simulink model "vienna_rectifier"  (R2026b)
settings: Solver=ode23tb  StopTime=param.sim.simlength  FixedStep=param.glb_time.tc  MaxStep=param.glb_time.tc
values from neighbouring files (symbols this model uses):
  param = struct()    [init_model.m]
undefined symbols (not defined in the file or in its folder): magnitude
libraries: fl_lib x42, nesl_utility x28, discrete_time_low_pass_filter x5, single_phase_transformer_lib x3, threephase_inductor_lib x1, dclink_for_three_levels x1, vienna_rectifier_ideal_switch_based_model x1, three_phase_three_levels_PWM_modulator x1, three_phase_voltage_with_frt_emulator x1
(part 3 of 4)

== system vienna_rectifier/afe_dq_mod1/AFE_control/afe_control/current_ctrl/zero_current_ctrl/zero_sequence_current_ctrl ==
  iz : Inport
  1/Ti : Gain  Gain=param.afe.ctrl.kp_is_z  SaturateOnIntegerOverflow=on  OutDataTypeStr=Inherit: Same as input  ParamDataTypeStr=Inherit: Same as input
  Constant1 : Constant  Value=0
  Gain : Gain
  Saturation : Saturate  UpperLimit=1  LowerLimit=-1
  Sum1 : Sum  Inputs=+++  SaturateOnIntegerOverflow=on
  Sum2 : Sum  Inputs=-+  SaturateOnIntegerOverflow=on
  Sum3 : Sum  Inputs=-+  SaturateOnIntegerOverflow=on
  Unit Delay4 : UnitDelay  SampleTime=-1
  iz_tracking : Scope  NumInputPorts=3
      settings: ActiveDisplayYMinimum=-1  ActiveDisplayYMaximum=1  DataLoggingVariableName=ScopeData8
  kp : Gain  Gain=param.afe.ctrl.ki_is_z*param.glb_time.ts_afe  SaturateOnIntegerOverflow=on  OutDataTypeStr=Inherit: Same as input  ParamDataTypeStr=Inherit: Same as input
  ugamma_afe : Outport
  tag scope: iz_ctrl_out=scoped, iz_pu=scoped, iz_pu_ref=scoped
  wires:
  1/Ti/1 -> Sum1/1, Sum3/1
  kp/1 -> Sum1/2
  Sum3/1 -> Unit Delay4/1
  Unit Delay4/1 -> Sum1/3
  Constant1/1 -> [iz_pu_ref], iz_tracking/1, Sum2/2  "iz_pu_ref"
  iz/1 -> [iz_pu], iz_tracking/2, Sum2/1  "iz_pu"
  Sum2/1 -> kp/1, 1/Ti/1
  Sum1/1 -> Saturation/1
  Saturation/1 -> Gain/1, [iz_ctrl_out], iz_tracking/3, Sum3/2  "iz_ctrl_out"
  Gain/1 -> ugamma_afe/1

== system vienna_rectifier/afe_dq_mod1/AFE_control/afe_control/grid_voltage_phase_lock_loops/DDSRF-PLL/pll_stageA ==
  gamma_grid : Inport
  ug_abc_pu : Inport  Port=2
  Demux : Demux  Outputs=3
  Math Function : Math  Operator=magnitude^2  SignedPower=on
  Math Function1 : Math  Operator=magnitude^2  SignedPower=on
  Reciprocal Sqrt : Sqrt  Operator=rSqrt
  Saturation : Saturate  UpperLimit=inf  LowerLimit=0.02
  Sum : Sum  Inputs=|++
  filter_and_transformation : Subsystem
  sequences : Subsystem
  u_grid_pos_xi : Outport  VectorParamsAs1DForOutWhenUnconnected=off
  u_grid_pos_eta : Outport  Port=2  VectorParamsAs1DForOutWhenUnconnected=off
  tag scope: Vgrid_unorm_ddsrf=scoped
  wires:
  Saturation/1 -> Reciprocal Sqrt/1
  Reciprocal Sqrt/1 -> [Vgrid_unorm_ddsrf]
  Sum/1 -> Saturation/1
  Math Function1/1 -> Sum/2
  Math Function/1 -> Sum/1
  filter_and_transformation/2(ug_beta) -> Math Function1/1, sequences/2(u_grid_beta)
  filter_and_transformation/1(ug_alpha) -> Math Function/1, sequences/1(u_grid_alpha)
  Demux/3 -> filter_and_transformation/3(ug_c)
  Demux/2 -> filter_and_transformation/2(ug_b)
  Demux/1 -> filter_and_transformation/1(ug_a)
  ug_abc_pu/1 -> Demux/1
  sequences/1(u_grid_pos_xi) -> u_grid_pos_xi/1
  sequences/2(u_grid_pos_eta) -> u_grid_pos_eta/1
  gamma_grid/1 -> sequences/3(phase_angle)

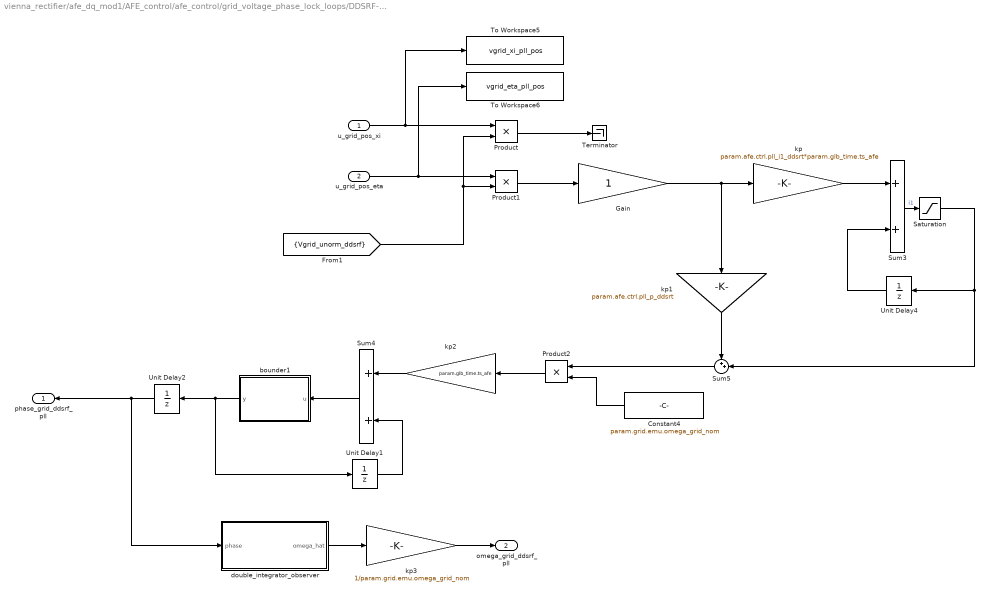
== system vienna_rectifier/afe_dq_mod1/AFE_control/afe_control/grid_voltage_phase_lock_loops/DDSRF-PLL/pll_stageB ==
  u_grid_pos_xi : Inport
  u_grid_pos_eta : Inport  Port=2
  Constant4 : Constant  Value=param.grid.emu.omega_grid_nom
  Gain : Gain
  Product : Product  RndMeth=Zero
  Product1 : Product  RndMeth=Zero
  Product2 : Product  RndMeth=Zero
  Saturation : Saturate  UpperLimit=1.5  LowerLimit=0.5
  Sum3 : Sum  SaturateOnIntegerOverflow=on
  Sum4 : Sum  SaturateOnIntegerOverflow=on
  Sum5 : Sum  Inputs=++|
  Terminator : Terminator
  To Workspace5 : ToWorkspace  VariableName=vgrid_xi_pll_pos  SampleTime=-1
      settings: MaxDataPoints=param.glb_time.Ns_afe
  To Workspace6 : ToWorkspace  VariableName=vgrid_eta_pll_pos  SampleTime=-1
      settings: MaxDataPoints=param.glb_time.Ns_afe
  Unit Delay1 : UnitDelay  SampleTime=-1
  Unit Delay2 : UnitDelay  SampleTime=-1
  Unit Delay4 : UnitDelay  InitialCondition=param.afe.pll.integrator_init  SampleTime=-1
  bounder1 : MATLAB Function  TreatAsAtomicUnit=on
  double_integrator_observer : Subsystem
  kp : Gain  Gain=param.afe.ctrl.pll_i1_ddsrt*param.glb_time.ts_afe  SaturateOnIntegerOverflow=on  OutDataTypeStr=Inherit: Same as input  ParamDataTypeStr=Inherit: Same as input
  kp1 : Gain  Gain=param.afe.ctrl.pll_p_ddsrt  SaturateOnIntegerOverflow=on  OutDataTypeStr=Inherit: Same as input  ParamDataTypeStr=Inherit: Same as input
  kp2 : Gain  Gain=param.glb_time.ts_afe  SaturateOnIntegerOverflow=on  OutDataTypeStr=Inherit: Same as input  ParamDataTypeStr=Inherit: Same as input
  kp3 : Gain  Gain=1/param.grid.emu.omega_grid_nom  SaturateOnIntegerOverflow=on  OutDataTypeStr=Inherit: Same as input  ParamDataTypeStr=Inherit: Same as input
  phase_grid_ddsrf_pll : Outport  VectorParamsAs1DForOutWhenUnconnected=off
  omega_grid_ddsrf_pll : Outport  Port=2  VectorParamsAs1DForOutWhenUnconnected=off
  wires:
  Unit Delay2/1 -> double_integrator_observer/1(phase), phase_grid_ddsrf_pll/1
  kp1/1 -> Sum5/1
  Product2/1 -> kp2/1
  u_grid_pos_eta/1 -> Product1/1, To Workspace6/1
  u_grid_pos_xi/1 -> To Workspace5/1, Product/1
  bounder1/1(y) -> Unit Delay1/1, Unit Delay2/1
  Sum5/1 -> Product2/1
  kp/1 -> Sum3/1
  [Vgrid_unorm_ddsrf] -> Product1/2, Product/2
  Constant4/1 -> Product2/2
  kp2/1 -> Sum4/1
  Sum3/1 -> Saturation/1  "i1"
  Saturation/1 -> Unit Delay4/1, Sum5/2
  Unit Delay1/1 -> Sum4/2
  Sum4/1 -> bounder1/1(u)
  Unit Delay4/1 -> Sum3/2
  double_integrator_observer/1(omega_hat) -> kp3/1
  Product/1 -> Terminator/1
  kp3/1 -> omega_grid_ddsrf_pll/1
  Product1/1 -> Gain/1
  Gain/1 -> kp1/1, kp/1

== system vienna_rectifier/afe_dq_mod1/AFE_control/afe_control/acquisitions/phase_compensation_1/alignment_eval_afe1/pi ==
  u_ref : Inport
  u : Inport  Port=2
  1/Ti : Gain  Gain=kp  SaturateOnIntegerOverflow=on  OutDataTypeStr=Inherit: Same as input  ParamDataTypeStr=Inherit: Same as input
  Saturation : Saturate  UpperLimit=lim_up  LowerLimit=lim_down
  Sum1 : Sum  Inputs=+++  SaturateOnIntegerOverflow=on
  Sum2 : Sum  Inputs=-+  SaturateOnIntegerOverflow=on
  Sum3 : Sum  Inputs=-+  SaturateOnIntegerOverflow=on
  Unit Delay4 : UnitDelay  SampleTime=-1
  kp : Gain  Gain=ki  SaturateOnIntegerOverflow=on  OutDataTypeStr=Inherit: Same as input  ParamDataTypeStr=Inherit: Same as input
  y : Outport
  wires:
  1/Ti/1 -> Sum1/1, Sum3/1
  kp/1 -> Sum1/2
  Sum3/1 -> Unit Delay4/1
  Unit Delay4/1 -> Sum1/3
  u_ref/1 -> Sum2/2
  u/1 -> Sum2/1
  Sum2/1 -> kp/1, 1/Ti/1
  Sum1/1 -> Saturation/1
  Saturation/1 -> Sum3/2, y/1

== system vienna_rectifier/afe_dq_mod1/AFE_control/afe_control/grid_voltage_phase_lock_loops/DDSRF-PLL/pll_stageA/filter_and_transformation ==
  ug_a : Inport
  ug_b : Inport  Port=2
  ug_c : Inport  Port=3
  abc2alphabeta : MATLAB Function  TreatAsAtomicUnit=on
  first_harmonic_tracker : Scope  NumInputPorts=3
      settings: ActiveDisplayYMinimum=-1.2482939809560776  ActiveDisplayYMaximum=1.2484282106161118  DataLoggingVariableName=ScopeData3
  first_harmonic_tracker_phase_u : Subsystem
  first_harmonic_tracker_phase_v : Subsystem
  first_harmonic_tracker_phase_w : Subsystem
  ug_alpha : Outport  VectorParamsAs1DForOutWhenUnconnected=off
  ug_beta : Outport  Port=2  VectorParamsAs1DForOutWhenUnconnected=off
  wires:
  abc2alphabeta/1(alpha) -> ug_alpha/1  "u_grid_alpha"
  abc2alphabeta/2(beta) -> ug_beta/1  "u_grid_beta"
  first_harmonic_tracker_phase_u/1(u_hat) -> first_harmonic_tracker/1, abc2alphabeta/1(a)  "tracker_phase_u"
  first_harmonic_tracker_phase_w/1(u_hat) -> first_harmonic_tracker/3, abc2alphabeta/3(c)  "tracker_phase_w"
  first_harmonic_tracker_phase_v/1(u_hat) -> first_harmonic_tracker/2, abc2alphabeta/2(b)  "tracker_phase_v"
  ug_a/1 -> first_harmonic_tracker_phase_u/1(u)
  ug_b/1 -> first_harmonic_tracker_phase_v/1(u)
  ug_c/1 -> first_harmonic_tracker_phase_w/1(u)

== system vienna_rectifier/afe_dq_mod1/AFE_control/afe_control/grid_voltage_phase_lock_loops/DDSRF-PLL/pll_stageA/sequences ==
  u_grid_alpha : Inport
  u_grid_beta : Inport  Port=2
  phase_angle : Inport  Port=3
  ddsrf : Subsystem
  u_grid_pos_xi : Outport
  u_grid_pos_eta : Outport  Port=2
  wires:
  phase_angle/1 -> ddsrf/3(phase_angle)  "phase_angle"
  u_grid_beta/1 -> ddsrf/2(u_grid_beta)  "u_grid_beta"
  u_grid_alpha/1 -> ddsrf/1(u_grid_alpha)  "u_grid_alpha"
  ddsrf/2(u_grid_pos_eta) -> u_grid_pos_eta/1  "u_grid_pos_eta"
  ddsrf/1(u_grid_pos_xi) -> u_grid_pos_xi/1  "u_grid_pos_xi"

== system vienna_rectifier/afe_dq_mod1/AFE_control/afe_control/grid_voltage_phase_lock_loops/DDSRF-PLL/pll_stageB/double_integrator_observer ==
  phase : Inport
  Gain : Gain  Gain=param.afe.ctrl.di_obs.Ldso  Multiplication=Matrix(K*u)
  Gain1 : Gain  Gain=param.afe.ctrl.di_obs.Adso  Multiplication=Matrix(K*u)
  Gain2 : Gain  Gain=param.afe.ctrl.di_obs.Cso  Multiplication=Matrix(K*u)
  Selector : Selector  InputPortWidth=2  IndexOptions=Index vector (dialog)  Indices=2  OutputSizes=1  RuntimeRangeChecks=off
  Sum : Sum  Inputs=-+|
  Sum1 : Sum  Inputs=|++
  Unit Delay : UnitDelay  SampleTime=-1
  bounder1 : MATLAB Function  TreatAsAtomicUnit=on
  bounder2 : MATLAB Function  TreatAsAtomicUnit=on
  omega_hat : Outport
  wires:
  Gain/1 -> Sum1/1
  Selector/1 -> omega_hat/1
  Gain2/1 -> bounder2/1(u)  "theta_hat"
  Gain1/1 -> Sum1/2
  Sum1/1 -> Unit Delay/1
  Sum/1 -> bounder1/1(u)  "e"
  Unit Delay/1 -> Gain1/1, Selector/1, Gain2/1
  phase/1 -> Sum/2  "phase"
  bounder1/1(y) -> Gain/1  "e_bounded"
  bounder2/1(y) -> Sum/1  "theta_hat_bounded"

== system vienna_rectifier/afe_dq_mod1/AFE_control/afe_control/grid_voltage_phase_lock_loops/DDSRF-PLL/pll_stageA/filter_and_transformation/first_harmonic_tracker_phase_u ==
  u : Inport
  Bus Selector : BusSelector  OutputSignals=output_pu_hat
  C Caller : CCaller  FunctionName=first_harmonic_tracker_process_simulink  PortSpecificationStruct="%)30     .    B \\   8    (     @         %    \"     D    !     0         %  0 \"0    $    _    07)G3F%M90  4&]R=$YA;64 4V-O<&4     26YD97@     5'EP90      4VEZ90      27-';&]B86P   X    P    !@    @    $          4    (     0    ,    !         !   P!O=70 #@   #     &    \"     0         !0    @    !     P    $         $  # &]U=  .    .     8    (    !          %    \"     $    &     0         0  ...(+4988 chars)"
  Constant : Constant  Value=param.glb_time.ts_afe
  Constant1 : Constant  Value=6
  Constant4 : Constant  Value=param.afe.ctrl.fht_grid.omega_fht
  Constant5 : Constant  Value=param.afe.ctrl.fht_grid.delta_fht
  Constant6 : Constant  Value=param.afe.ctrl.fht_grid.Ld_fht(1)
  Constant7 : Constant  Value=param.afe.ctrl.fht_grid.Ld_fht(2)
  Data Type Conversion{1..2,6..9} (6 alike) : DataTypeConversion  OutDataTypeStr=single  SaturateOnIntegerOverflow=off  RndMeth=Floor
  Data Type Conversion3 : DataTypeConversion  OutDataTypeStr=uint8  SaturateOnIntegerOverflow=off  RndMeth=Floor
  Data Type Conversion4 : DataTypeConversion  OutDataTypeStr=double  SaturateOnIntegerOverflow=off  RndMeth=Floor
  Data Type Conversion5 : DataTypeConversion  OutDataTypeStr=uint8  SaturateOnIntegerOverflow=off  RndMeth=Floor
  Step : Step  Time=0.0125  InitialValue=1  FinalValue=0
  u_hat : Outport
  wires:
  Data Type Conversion4/1 -> u_hat/1
  Data Type Conversion3/1 -> C Caller/1
  Data Type Conversion1/1 -> C Caller/3
  Data Type Conversion2/1 -> C Caller/2
  C Caller/1 -> Bus Selector/1
  Bus Selector/1 -> Data Type Conversion4/1  "<output_pu_hat>"
  Step/1 -> Data Type Conversion3/1
  u/1 -> Data Type Conversion2/1
  Constant/1 -> Data Type Conversion1/1
  Constant1/1 -> Data Type Conversion5/1
  Constant4/1 -> Data Type Conversion6/1
  Constant6/1 -> Data Type Conversion8/1
  Constant7/1 -> Data Type Conversion9/1
  Constant5/1 -> Data Type Conversion7/1
  Data Type Conversion5/1 -> C Caller/8
  Data Type Conversion6/1 -> C Caller/4
  Data Type Conversion7/1 -> C Caller/5
  Data Type Conversion8/1 -> C Caller/6
  Data Type Conversion9/1 -> C Caller/7

== system vienna_rectifier/afe_dq_mod1/AFE_control/afe_control/grid_voltage_phase_lock_loops/DDSRF-PLL/pll_stageA/filter_and_transformation/first_harmonic_tracker_phase_v ==
  u : Inport
  Bus Selector : BusSelector  OutputSignals=output_pu_hat
  C Caller : CCaller  FunctionName=first_harmonic_tracker_process_simulink  PortSpecificationStruct="%)30     .    B \\   8    (     @         %    \"     D    !     0         %  0 \"0    $    _    07)G3F%M90  4&]R=$YA;64 4V-O<&4     26YD97@     5'EP90      4VEZ90      27-';&]B86P   X    P    !@    @    $          4    (     0    ,    !         !   P!O=70 #@   #     &    \"     0         !0    @    !     P    $         $  # &]U=  .    .     8    (    !          %    \"     $    &     0         0  ...(+4988 chars)"
  Constant : Constant  Value=param.glb_time.ts_afe
  Constant1 : Constant  Value=8
  Constant4 : Constant  Value=param.afe.ctrl.fht_grid.omega_fht
  Constant5 : Constant  Value=param.afe.ctrl.fht_grid.delta_fht
  Constant6 : Constant  Value=param.afe.ctrl.fht_grid.Ld_fht(1)
  Constant7 : Constant  Value=param.afe.ctrl.fht_grid.Ld_fht(2)
  Data Type Conversion{1..2,6..9} (6 alike) : DataTypeConversion  OutDataTypeStr=single  SaturateOnIntegerOverflow=off  RndMeth=Floor
  Data Type Conversion3 : DataTypeConversion  OutDataTypeStr=uint8  SaturateOnIntegerOverflow=off  RndMeth=Floor
  Data Type Conversion4 : DataTypeConversion  OutDataTypeStr=double  SaturateOnIntegerOverflow=off  RndMeth=Floor
  Data Type Conversion5 : DataTypeConversion  OutDataTypeStr=uint8  SaturateOnIntegerOverflow=off  RndMeth=Floor
  Step : Step  Time=0.0125  InitialValue=1  FinalValue=0
  u_hat : Outport
  wires:
  Data Type Conversion9/1 -> C Caller/7
  Data Type Conversion8/1 -> C Caller/6
  Data Type Conversion7/1 -> C Caller/5
  Data Type Conversion6/1 -> C Caller/4
  Data Type Conversion5/1 -> C Caller/8
  Constant5/1 -> Data Type Conversion7/1
  Constant7/1 -> Data Type Conversion9/1
  Constant6/1 -> Data Type Conversion8/1
  Constant4/1 -> Data Type Conversion6/1
  Constant1/1 -> Data Type Conversion5/1
  Constant/1 -> Data Type Conversion1/1
  u/1 -> Data Type Conversion2/1
  Step/1 -> Data Type Conversion3/1
  Bus Selector/1 -> Data Type Conversion4/1  "<output_pu_hat>"
  C Caller/1 -> Bus Selector/1
  Data Type Conversion2/1 -> C Caller/2
  Data Type Conversion1/1 -> C Caller/3
  Data Type Conversion3/1 -> C Caller/1
  Data Type Conversion4/1 -> u_hat/1

== system vienna_rectifier/afe_dq_mod1/AFE_control/afe_control/grid_voltage_phase_lock_loops/DDSRF-PLL/pll_stageA/filter_and_transformation/first_harmonic_tracker_phase_w ==
  u : Inport
  Bus Selector : BusSelector  OutputSignals=output_pu_hat
  C Caller : CCaller  FunctionName=first_harmonic_tracker_process_simulink  PortSpecificationStruct="%)30     .    B \\   8    (     @         %    \"     D    !     0         %  0 \"0    $    _    07)G3F%M90  4&]R=$YA;64 4V-O<&4     26YD97@     5'EP90      4VEZ90      27-';&]B86P   X    P    !@    @    $          4    (     0    ,    !         !   P!O=70 #@   #     &    \"     0         !0    @    !     P    $         $  # &]U=  .    .     8    (    !          %    \"     $    &     0         0  ...(+4988 chars)"
  Constant : Constant  Value=param.glb_time.ts_afe
  Constant1 : Constant  Value=10
  Constant4 : Constant  Value=param.afe.ctrl.fht_grid.omega_fht
  Constant5 : Constant  Value=param.afe.ctrl.fht_grid.delta_fht
  Constant6 : Constant  Value=param.afe.ctrl.fht_grid.Ld_fht(1)
  Constant7 : Constant  Value=param.afe.ctrl.fht_grid.Ld_fht(2)
  Data Type Conversion{1..2,6..9} (6 alike) : DataTypeConversion  OutDataTypeStr=single  SaturateOnIntegerOverflow=off  RndMeth=Floor
  Data Type Conversion3 : DataTypeConversion  OutDataTypeStr=uint8  SaturateOnIntegerOverflow=off  RndMeth=Floor
  Data Type Conversion4 : DataTypeConversion  OutDataTypeStr=double  SaturateOnIntegerOverflow=off  RndMeth=Floor
  Data Type Conversion5 : DataTypeConversion  OutDataTypeStr=uint8  SaturateOnIntegerOverflow=off  RndMeth=Floor
  Step : Step  Time=0.0125  InitialValue=1  FinalValue=0
  u_hat : Outport
  wires:
  Data Type Conversion4/1 -> u_hat/1
  Data Type Conversion3/1 -> C Caller/1
  Data Type Conversion1/1 -> C Caller/3
  Data Type Conversion2/1 -> C Caller/2
  C Caller/1 -> Bus Selector/1
  Bus Selector/1 -> Data Type Conversion4/1  "<output_pu_hat>"
  Step/1 -> Data Type Conversion3/1
  u/1 -> Data Type Conversion2/1
  Constant/1 -> Data Type Conversion1/1
  Constant1/1 -> Data Type Conversion5/1
  Constant4/1 -> Data Type Conversion6/1
  Constant6/1 -> Data Type Conversion8/1
  Constant7/1 -> Data Type Conversion9/1
  Constant5/1 -> Data Type Conversion7/1
  Data Type Conversion5/1 -> C Caller/8
  Data Type Conversion6/1 -> C Caller/4
  Data Type Conversion7/1 -> C Caller/5
  Data Type Conversion8/1 -> C Caller/6
  Data Type Conversion9/1 -> C Caller/7

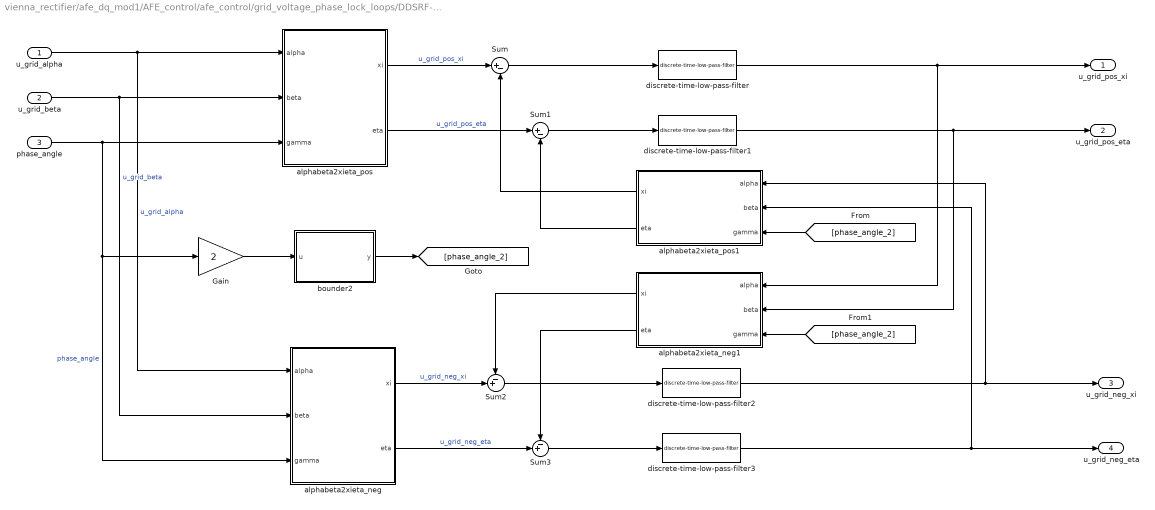
== system vienna_rectifier/afe_dq_mod1/AFE_control/afe_control/grid_voltage_phase_lock_loops/DDSRF-PLL/pll_stageA/sequences/ddsrf ==
  u_grid_alpha : Inport
  u_grid_beta : Inport  Port=2
  phase_angle : Inport  Port=3
  Gain : Gain  Gain=2
  Sum : Sum  Inputs=|+-
  Sum1 : Sum  Inputs=|+-
  Sum2 : Sum  Inputs=-+|
  Sum3 : Sum  Inputs=-+|
  alphabeta2xieta_neg : MATLAB Function  TreatAsAtomicUnit=on
  alphabeta2xieta_neg1 : MATLAB Function  TreatAsAtomicUnit=on
  alphabeta2xieta_pos : MATLAB Function  TreatAsAtomicUnit=on
  alphabeta2xieta_pos1 : MATLAB Function  TreatAsAtomicUnit=on
  bounder2 : MATLAB Function  TreatAsAtomicUnit=on
  discrete-time-low-pass-filter{,1..3} (4 alike) : discrete_time_low_pass_filter/discrete-time-low-pass-filter  tau=param.afe.ctrl.tau_ddsrf  ts=param.glb_time.ts_afe
  u_grid_pos_xi : Outport
  u_grid_pos_eta : Outport  Port=2
  u_grid_neg_xi : Outport  Port=3
  u_grid_neg_eta : Outport  Port=4
  wires:
  phase_angle/1 -> alphabeta2xieta_pos/3(gamma), alphabeta2xieta_neg/3(gamma), Gain/1  "phase_angle"
  u_grid_beta/1 -> alphabeta2xieta_pos/2(beta), alphabeta2xieta_neg/2(beta)  "u_grid_beta"
  u_grid_alpha/1 -> alphabeta2xieta_pos/1(alpha), alphabeta2xieta_neg/1(alpha)  "u_grid_alpha"
  alphabeta2xieta_pos/1(xi) -> Sum/1  "u_grid_pos_xi"
  Sum/1 -> discrete-time-low-pass-filter/1
  alphabeta2xieta_pos/2(eta) -> Sum1/1  "u_grid_pos_eta"
  Sum1/1 -> discrete-time-low-pass-filter1/1
  alphabeta2xieta_neg/1(xi) -> Sum2/2  "u_grid_neg_xi"
  Sum2/1 -> discrete-time-low-pass-filter2/1
  Sum3/1 -> discrete-time-low-pass-filter3/1
  alphabeta2xieta_neg/2(eta) -> Sum3/2  "u_grid_neg_eta"
  Gain/1 -> bounder2/1(u)
  discrete-time-low-pass-filter/1 -> u_grid_pos_xi/1, alphabeta2xieta_neg1/1(alpha)
  discrete-time-low-pass-filter1/1 -> u_grid_pos_eta/1, alphabeta2xieta_neg1/2(beta)
  discrete-time-low-pass-filter2/1 -> u_grid_neg_xi/1, alphabeta2xieta_pos1/1(alpha)
  discrete-time-low-pass-filter3/1 -> u_grid_neg_eta/1, alphabeta2xieta_pos1/2(beta)
  bounder2/1(y) -> [phase_angle_2]
  [phase_angle_2] -> alphabeta2xieta_pos1/3(gamma)
  [phase_angle_2] -> alphabeta2xieta_neg1/3(gamma)
  alphabeta2xieta_pos1/1(xi) -> Sum/2
  alphabeta2xieta_pos1/2(eta) -> Sum1/2
  alphabeta2xieta_neg1/1(xi) -> Sum2/1
  alphabeta2xieta_neg1/2(eta) -> Sum3/1

== matlab function vienna_rectifier/afe_dq_mod1/AFE_control/afe_control/current_ctrl/xi_eta_to_alpha_beta ==
  data: xi input; alpha output; eta input; phase input; beta output
function [alpha,beta] = xi_eta_to_alpha_beta(xi,eta,phase)

    alpha = xi*cos(phase) - eta*sin(phase);
    beta  = xi*sin(phase) + eta*cos(phase);

end

== matlab function vienna_rectifier/afe_dq_mod1/AFE_control/afe_control/grid_voltage_phase_lock_loops/DDSRF-PLL/pll_stageA/sequences/ddsrf/alphabeta2xieta_neg1 ==
  data: alpha input; xi output; beta input; gamma input; eta output
function [xi,eta] = alphabeta2xieta_neg(alpha,beta,gamma)

    xi  = alpha*cos(gamma) - beta*sin(gamma);
    eta = alpha*sin(gamma) + beta*cos(gamma);

end

== matlab function vienna_rectifier/afe_dq_mod1/AFE_control/afe_control/grid_voltage_phase_lock_loops/DDSRF-PLL/pll_stageA/sequences/ddsrf/alphabeta2xieta_pos ==
  data: alpha input; xi output; beta input; gamma input; eta output
function [xi,eta] = alphabeta2xieta_pos(alpha,beta,gamma)

    xi  =  alpha*cos(gamma) + beta*sin(gamma);
    eta = -alpha*sin(gamma) + beta*cos(gamma);

end

== matlab function vienna_rectifier/afe_dq_mod1/AFE_control/afe_control/grid_voltage_phase_lock_loops/DDSRF-PLL/pll_stageA/sequences/ddsrf/alphabeta2xieta_pos1 ==
  data: alpha input; xi output; beta input; gamma input; eta output
function [xi,eta] = alphabeta2xieta_pos(alpha,beta,gamma)

    xi  =  alpha*cos(gamma) + beta*sin(gamma);
    eta = -alpha*sin(gamma) + beta*cos(gamma);

end

== matlab function vienna_rectifier/afe_dq_mod1/AFE_control/afe_control/grid_voltage_phase_lock_loops/DDSRF-PLL/pll_stageA/sequences/ddsrf/bounder2 ==
  data: u input; y output
function y = bounder(u)
    
    y = -pi + mod(u+3*pi,2*pi);
    % y = mod(u, 2*pi);
    
end

== matlab function vienna_rectifier/afe_dq_mod1/AFE_control/afe_control/grid_voltage_phase_lock_loops/DDSRF-PLL/pll_stageB/bounder1 ==
  data: u input; y output
function y = bounder(u)
    y = -pi + mod(u+3*pi,2*pi);
end

== matlab function vienna_rectifier/afe_dq_mod1/rectifier/deadtime_generator_for_ttype/dead_time_generator_cmos_simulink_phu/dead_time_leg_generator_1/MATLAB Function ==
  data: u input; y output; Vpos_rail_dtg parameter
function y = not_cmos(u, Vpos_rail_dtg)

vth = Vpos_rail_dtg/2;

if u > vth
    y = 0;
else
    y = Vpos_rail_dtg;
end

== matlab function vienna_rectifier/afe_dq_mod1/rectifier/deadtime_generator_for_ttype/dead_time_generator_cmos_simulink_phu/dead_time_leg_generator_1/MATLAB Function1 ==
  data: u1 input; u2 input; y output; Vpos_rail_dtg parameter
function y = and_cmos(u1, u2, Vpos_rail_dtg)

vth = Vpos_rail_dtg/2;

if (u1 > vth && u2 > vth)
    y = Vpos_rail_dtg;
else
    y = 0;
end

== matlab function vienna_rectifier/afe_dq_mod1/rectifier/deadtime_generator_for_ttype/dead_time_generator_cmos_simulink_phu/dead_time_leg_generator_1/MATLAB Function2 ==
  data: u input; y output; Vpos_rail_dtg parameter
function y = not_cmos(u, Vpos_rail_dtg)

vth = Vpos_rail_dtg/2;

if u > vth
    y = 0;
else
    y = Vpos_rail_dtg;
end

== matlab function vienna_rectifier/afe_dq_mod1/rectifier/deadtime_generator_for_ttype/dead_time_generator_cmos_simulink_phu/dead_time_leg_generator_1/MATLAB Function3 ==
  data: u input; y output; Vpos_rail_dtg parameter
function y = not_cmos(u, Vpos_rail_dtg)

vth = Vpos_rail_dtg/2;

if u > vth
    y = 0;
else
    y = Vpos_rail_dtg;
end

== matlab function vienna_rectifier/afe_dq_mod1/rectifier/deadtime_generator_for_ttype/dead_time_generator_cmos_simulink_phu/dead_time_leg_generator_1/MATLAB Function4 ==
  data: u1 input; u2 input; y output; Vpos_rail_dtg parameter
function y = and_cmos(u1, u2, Vpos_rail_dtg)

vth = Vpos_rail_dtg/2;

if (u1 > vth && u2 > vth)
    y = Vpos_rail_dtg;
else
    y = 0;
end

== matlab function vienna_rectifier/afe_dq_mod1/rectifier/deadtime_generator_for_ttype/dead_time_generator_cmos_simulink_phu/dead_time_leg_generator_1/MATLAB Function5 ==
  data: u1 input; u2 input; y output; Vpos_rail_dtg parameter
function y = and_cmos(u1, u2, Vpos_rail_dtg)

vth = Vpos_rail_dtg/2;

if (u1 > vth && u2 > vth)
    y = Vpos_rail_dtg;
else
    y = 0;
end

== matlab function vienna_rectifier/afe_dq_mod1/rectifier/deadtime_generator_for_ttype/dead_time_generator_cmos_simulink_phu/dead_time_leg_generator_1/MATLAB Function6 ==
  data: u input; y output; Vpos_rail_dtg parameter
function y = not_cmos(u, Vpos_rail_dtg)

vth = Vpos_rail_dtg/2;

if u > vth
    y = 0;
else
    y = Vpos_rail_dtg;
end

== matlab function vienna_rectifier/afe_dq_mod1/rectifier/deadtime_generator_for_ttype/dead_time_generator_cmos_simulink_phu/dead_time_leg_generator_1/MATLAB Function7 ==
  data: u input; y output; Vpos_rail_dtg parameter
function y = not_cmos(u, Vpos_rail_dtg)

vth = Vpos_rail_dtg/2;

if u > vth
    y = 0;
else
    y = Vpos_rail_dtg;
end

== matlab function vienna_rectifier/afe_dq_mod1/rectifier/deadtime_generator_for_ttype/dead_time_generator_cmos_simulink_phu/dead_time_leg_generator_1/MATLAB Function8 ==
  data: u input; y output; Vpos_rail_dtg parameter
function y = not_cmos(u, Vpos_rail_dtg)

vth = Vpos_rail_dtg/2;

if u > vth
    y = 0;
else
    y = Vpos_rail_dtg;
end

== matlab function vienna_rectifier/afe_dq_mod1/rectifier/deadtime_generator_for_ttype/dead_time_generator_cmos_simulink_phu/dead_time_leg_generator_1/MATLAB Function9 ==
  data: u1 input; u2 input; y output; Vpos_rail_dtg parameter
function y = and_cmos(u1, u2, Vpos_rail_dtg)

vth = Vpos_rail_dtg/2;

if (u1 > vth && u2 > vth)
    y = Vpos_rail_dtg;
else
    y = 0;
end

== matlab function vienna_rectifier/afe_dq_mod1/rectifier/deadtime_generator_for_ttype/dead_time_generator_cmos_simulink_phv/dead_time_leg_generator_1/MATLAB Function ==
  data: u input; y output; Vpos_rail_dtg parameter
function y = not_cmos(u, Vpos_rail_dtg)

vth = Vpos_rail_dtg/2;

if u > vth
    y = 0;
else
    y = Vpos_rail_dtg;
end

== matlab function vienna_rectifier/afe_dq_mod1/rectifier/deadtime_generator_for_ttype/dead_time_generator_cmos_simulink_phv/dead_time_leg_generator_1/MATLAB Function1 ==
  data: u1 input; u2 input; y output; Vpos_rail_dtg parameter
function y = and_cmos(u1, u2, Vpos_rail_dtg)

vth = Vpos_rail_dtg/2;

if (u1 > vth && u2 > vth)
    y = Vpos_rail_dtg;
else
    y = 0;
end

== matlab function vienna_rectifier/afe_dq_mod1/rectifier/deadtime_generator_for_ttype/dead_time_generator_cmos_simulink_phv/dead_time_leg_generator_1/MATLAB Function2 ==
  data: u input; y output; Vpos_rail_dtg parameter
function y = not_cmos(u, Vpos_rail_dtg)

vth = Vpos_rail_dtg/2;

if u > vth
    y = 0;
else
    y = Vpos_rail_dtg;
end

== matlab function vienna_rectifier/afe_dq_mod1/rectifier/deadtime_generator_for_ttype/dead_time_generator_cmos_simulink_phv/dead_time_leg_generator_1/MATLAB Function3 ==
  data: u input; y output; Vpos_rail_dtg parameter
function y = not_cmos(u, Vpos_rail_dtg)

vth = Vpos_rail_dtg/2;

if u > vth
    y = 0;
else
    y = Vpos_rail_dtg;
end

== matlab function vienna_rectifier/afe_dq_mod1/rectifier/deadtime_generator_for_ttype/dead_time_generator_cmos_simulink_phv/dead_time_leg_generator_1/MATLAB Function4 ==
  data: u1 input; u2 input; y output; Vpos_rail_dtg parameter
function y = and_cmos(u1, u2, Vpos_rail_dtg)

vth = Vpos_rail_dtg/2;

if (u1 > vth && u2 > vth)
    y = Vpos_rail_dtg;
else
    y = 0;
end

== matlab function vienna_rectifier/afe_dq_mod1/rectifier/deadtime_generator_for_ttype/dead_time_generator_cmos_simulink_phv/dead_time_leg_generator_1/MATLAB Function5 ==
  data: u1 input; u2 input; y output; Vpos_rail_dtg parameter
function y = and_cmos(u1, u2, Vpos_rail_dtg)

vth = Vpos_rail_dtg/2;

if (u1 > vth && u2 > vth)
    y = Vpos_rail_dtg;
else
    y = 0;
end

== matlab function vienna_rectifier/afe_dq_mod1/rectifier/deadtime_generator_for_ttype/dead_time_generator_cmos_simulink_phv/dead_time_leg_generator_1/MATLAB Function6 ==
  data: u input; y output; Vpos_rail_dtg parameter
function y = not_cmos(u, Vpos_rail_dtg)

vth = Vpos_rail_dtg/2;

if u > vth
    y = 0;
else
    y = Vpos_rail_dtg;
end

== matlab function vienna_rectifier/afe_dq_mod1/rectifier/deadtime_generator_for_ttype/dead_time_generator_cmos_simulink_phv/dead_time_leg_generator_1/MATLAB Function7 ==
  data: u input; y output; Vpos_rail_dtg parameter
function y = not_cmos(u, Vpos_rail_dtg)

vth = Vpos_rail_dtg/2;

if u > vth
    y = 0;
else
    y = Vpos_rail_dtg;
end

== matlab function vienna_rectifier/afe_dq_mod1/rectifier/deadtime_generator_for_ttype/dead_time_generator_cmos_simulink_phv/dead_time_leg_generator_1/MATLAB Function8 ==
  data: u input; y output; Vpos_rail_dtg parameter
function y = not_cmos(u, Vpos_rail_dtg)

vth = Vpos_rail_dtg/2;

if u > vth
    y = 0;
else
    y = Vpos_rail_dtg;
end

== matlab function vienna_rectifier/afe_dq_mod1/rectifier/deadtime_generator_for_ttype/dead_time_generator_cmos_simulink_phv/dead_time_leg_generator_1/MATLAB Function9 ==
  data: u1 input; u2 input; y output; Vpos_rail_dtg parameter
function y = and_cmos(u1, u2, Vpos_rail_dtg)

vth = Vpos_rail_dtg/2;

if (u1 > vth && u2 > vth)
    y = Vpos_rail_dtg;
else
    y = 0;
end

== matlab function vienna_rectifier/afe_dq_mod1/rectifier/deadtime_generator_for_ttype/dead_time_generator_cmos_simulink_phw/dead_time_leg_generator_1/MATLAB Function ==
  data: u input; y output; Vpos_rail_dtg parameter
function y = not_cmos(u, Vpos_rail_dtg)

vth = Vpos_rail_dtg/2;

if u > vth
    y = 0;
else
    y = Vpos_rail_dtg;
end

== matlab function vienna_rectifier/afe_dq_mod1/rectifier/deadtime_generator_for_ttype/dead_time_generator_cmos_simulink_phw/dead_time_leg_generator_1/MATLAB Function1 ==
  data: u1 input; u2 input; y output; Vpos_rail_dtg parameter
function y = and_cmos(u1, u2, Vpos_rail_dtg)

vth = Vpos_rail_dtg/2;

if (u1 > vth && u2 > vth)
    y = Vpos_rail_dtg;
else
    y = 0;
end

== matlab function vienna_rectifier/afe_dq_mod1/rectifier/deadtime_generator_for_ttype/dead_time_generator_cmos_simulink_phw/dead_time_leg_generator_1/MATLAB Function2 ==
  data: u input; y output; Vpos_rail_dtg parameter
function y = not_cmos(u, Vpos_rail_dtg)

vth = Vpos_rail_dtg/2;

if u > vth
    y = 0;
else
    y = Vpos_rail_dtg;
end

== matlab function vienna_rectifier/afe_dq_mod1/rectifier/deadtime_generator_for_ttype/dead_time_generator_cmos_simulink_phw/dead_time_leg_generator_1/MATLAB Function3 ==
  data: u input; y output; Vpos_rail_dtg parameter
function y = not_cmos(u, Vpos_rail_dtg)

vth = Vpos_rail_dtg/2;

if u > vth
    y = 0;
else
    y = Vpos_rail_dtg;
end

== matlab function vienna_rectifier/afe_dq_mod1/rectifier/deadtime_generator_for_ttype/dead_time_generator_cmos_simulink_phw/dead_time_leg_generator_1/MATLAB Function4 ==
  data: u1 input; u2 input; y output; Vpos_rail_dtg parameter
function y = and_cmos(u1, u2, Vpos_rail_dtg)

vth = Vpos_rail_dtg/2;

if (u1 > vth && u2 > vth)
    y = Vpos_rail_dtg;
else
    y = 0;
end

== matlab function vienna_rectifier/afe_dq_mod1/rectifier/deadtime_generator_for_ttype/dead_time_generator_cmos_simulink_phw/dead_time_leg_generator_1/MATLAB Function5 ==
  data: u1 input; u2 input; y output; Vpos_rail_dtg parameter
function y = and_cmos(u1, u2, Vpos_rail_dtg)

vth = Vpos_rail_dtg/2;

if (u1 > vth && u2 > vth)
    y = Vpos_rail_dtg;
else
    y = 0;
end

== matlab function vienna_rectifier/afe_dq_mod1/rectifier/deadtime_generator_for_ttype/dead_time_generator_cmos_simulink_phw/dead_time_leg_generator_1/MATLAB Function6 ==
  data: u input; y output; Vpos_rail_dtg parameter
function y = not_cmos(u, Vpos_rail_dtg)

vth = Vpos_rail_dtg/2;

if u > vth
    y = 0;
else
    y = Vpos_rail_dtg;
end

== matlab function vienna_rectifier/afe_dq_mod1/rectifier/deadtime_generator_for_ttype/dead_time_generator_cmos_simulink_phw/dead_time_leg_generator_1/MATLAB Function7 ==
  data: u input; y output; Vpos_rail_dtg parameter
function y = not_cmos(u, Vpos_rail_dtg)

vth = Vpos_rail_dtg/2;

if u > vth
    y = 0;
else
    y = Vpos_rail_dtg;
end

== matlab function vienna_rectifier/afe_dq_mod1/rectifier/deadtime_generator_for_ttype/dead_time_generator_cmos_simulink_phw/dead_time_leg_generator_1/MATLAB Function8 ==
  data: u input; y output; Vpos_rail_dtg parameter
function y = not_cmos(u, Vpos_rail_dtg)

vth = Vpos_rail_dtg/2;

if u > vth
    y = 0;
else
    y = Vpos_rail_dtg;
end

== matlab function vienna_rectifier/afe_dq_mod1/rectifier/deadtime_generator_for_ttype/dead_time_generator_cmos_simulink_phw/dead_time_leg_generator_1/MATLAB Function9 ==
  data: u1 input; u2 input; y output; Vpos_rail_dtg parameter
function y = and_cmos(u1, u2, Vpos_rail_dtg)

vth = Vpos_rail_dtg/2;

if (u1 > vth && u2 > vth)
    y = Vpos_rail_dtg;
else
    y = 0;
end

== matlab function vienna_rectifier/afe_dq_mod1/AFE_control/afe_control/grid_voltage_phase_lock_loops/DDSRF-PLL/pll_stageB/double_integrator_observer/bounder1 ==
  data: u input; y output
function y = bounder(u)
    
    y = -pi + mod(u+3*pi,2*pi);
    
end

== matlab function vienna_rectifier/afe_dq_mod1/AFE_control/afe_control/grid_voltage_phase_lock_loops/DDSRF-PLL/pll_stageB/double_integrator_observer/bounder2 ==
  data: u input; y output
function y = bounder(u)
    
    y = -pi + mod(u+3*pi,2*pi);
    
end

== matlab function vienna_rectifier/afe_dq_mod1/AFE_control/afe_control/current_ctrl/current_transformation/uvw2alphabeta ==
  data: u input; alpha output; v input; w input; beta output
function [alpha,beta] = uvw2alphabeta(u,v,w)

alpha = 2/3*(u - 1/2*v - 1/2*w);
beta  = 2/3*(sqrt(3)/2*(v - w));

end

== matlab function vienna_rectifier/afe_dq_mod1/AFE_control/afe_control/current_ctrl/current_transformation/alphabeta2xieta ==
  data: alpha input; xi output; beta input; gamma input; eta output
function [xi,eta] = alphabeta2xieta(alpha,beta,gamma)

    xi  =  alpha*cos(gamma) + beta*sin(gamma);
    eta = -alpha*sin(gamma) + beta*cos(gamma);

end

== matlab function vienna_rectifier/afe_dq_mod1/AFE_control/afe_control/grid_voltage_phase_lock_loops/DDSRF-PLL/pll_stageA/filter_and_transformation/abc2alphabeta ==
  data: a input; alpha output; b input; c input; beta output
function [alpha,beta] = abc2alphabeta(a,b,c)

alpha = 2/3*(a - 1/2*b - 1/2*c);
beta  = 1/sqrt(3)*(b - c);

end

== matlab function vienna_rectifier/afe_dq_mod1/AFE_control/afe_control/grid_voltage_phase_lock_loops/DDSRF-PLL/pll_stageA/sequences/ddsrf/alphabeta2xieta_neg ==
  data: alpha input; xi output; beta input; gamma input; eta output
function [xi,eta] = alphabeta2xieta_neg(alpha,beta,gamma)

    xi  = alpha*cos(gamma) - beta*sin(gamma);
    eta = alpha*sin(gamma) + beta*cos(gamma);

end
